simulink model "UAV3_Safety_06"  (R2026b)
settings: Solver=FixedStepDiscrete  FixedStep=0.1
settings Model: Creator=Ivan  LastModifiedBy=Ivan

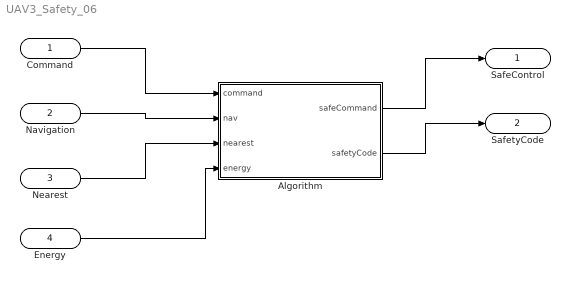
== system UAV3_Safety_06 ==
  Command : Inport  OutDataTypeStr=double  PortDimensions=[2 1]
  Navigation : Inport  Port=2  OutDataTypeStr=double  PortDimensions=[4 1]
  Nearest : Inport  Port=3  OutDataTypeStr=double  PortDimensions=[4 1]
  Energy : Inport  Port=4  OutDataTypeStr=double  PortDimensions=[3 1]
  Algorithm : MATLAB Function  TreatAsAtomicUnit=on
  SafeControl : Outport
  SafetyCode : Outport  Port=2
  wires:
  Command/1 -> Algorithm/1(command)
  Navigation/1 -> Algorithm/2(nav)
  Nearest/1 -> Algorithm/3(nearest)
  Energy/1 -> Algorithm/4(energy)
  Algorithm/1(safeCommand) -> SafeControl/1
  Algorithm/2(safetyCode) -> SafetyCode/1

== matlab function UAV3_Safety_06/Algorithm ==
  data: command input; safeCommand output; nav input; nearest input; energy input; safetyCode output
function [safeCommand,safetyCode] = v3_safety(command,nav,nearest,energy)
%V3_SAFETY Reactive brake/steer for threat or critical battery.
% Safety is a guard, not a mathematical safety guarantee.
% code 0=normal,1=avoid,2=low battery,3=invalid estimate.
%#codegen
safeCommand=command;
safetyCode=0.0;
if any(~isfinite(nav)) || any(~isfinite(command))
    safeCommand=zeros(2,1);
    safetyCode=3.0;
    return;
end
if energy(2)<=5.0
    safeCommand=-1.5*nav(3:4);
    safetyCode=2.0;
else
    r=nearest(2:3);
    d=nearest(1);
    speed2=dot(nav(3:4),nav(3:4));
    approach=0.0;
    if speed2>1e-9
        approach=max(0.0,min(2.0,dot(r,nav(3:4))/speed2));
    end
    prediction=sqrt(sum((r-approach*nav(3:4)).^2))-nearest(4);
    if d<4.0 || (approach>0.0 && prediction<4.0)
        away=-r-0.6*nav(3:4);
        m=sqrt(sum(away.^2));
        if m>1e-9
            safeCommand=3.0*away/m;
        else
            safeCommand=-1.5*nav(3:4);
        end
        safetyCode=1.0;
    end
end
a=sqrt(sum(safeCommand.^2));
if a>3.0
    safeCommand=3.0*safeCommand/a;
end
end
